simulink model "turbofan_engine_model"  (R2026b)
settings: Solver=ode45
settings Model: Creator=samjoseph  LastModifiedBy=samjoseph

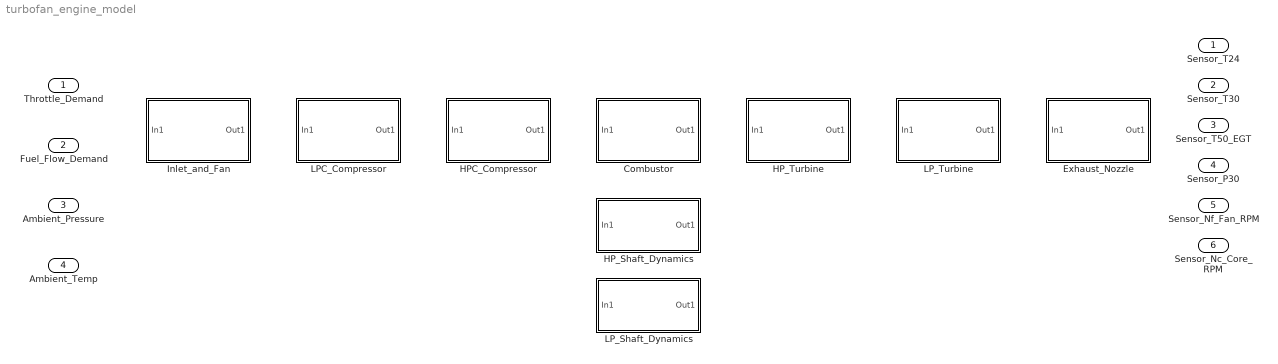
== system turbofan_engine_model ==
  Throttle_Demand : Inport
  Fuel_Flow_Demand : Inport  Port=2
  Ambient_Pressure : Inport  Port=3
  Ambient_Temp : Inport  Port=4
  Combustor : Subsystem
  Exhaust_Nozzle : Subsystem
  HPC_Compressor : Subsystem
  HP_Shaft_Dynamics : Subsystem
  HP_Turbine : Subsystem
  Inlet_and_Fan : Subsystem
  LPC_Compressor : Subsystem
  LP_Shaft_Dynamics : Subsystem
  LP_Turbine : Subsystem
  Sensor_T24 : Outport
  Sensor_T30 : Outport  Port=2
  Sensor_T50_EGT : Outport  Port=3
  Sensor_P30 : Outport  Port=4
  Sensor_Nf_Fan_RPM : Outport  Port=5
  Sensor_Nc_Core_RPM : Outport  Port=6

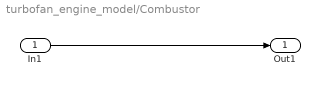
== system turbofan_engine_model/Combustor ==
  In1 : Inport
  Out1 : Outport
  wires:
  In1/1 -> Out1/1

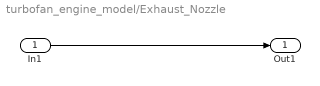
== system turbofan_engine_model/Exhaust_Nozzle ==
  In1 : Inport
  Out1 : Outport
  wires:
  In1/1 -> Out1/1

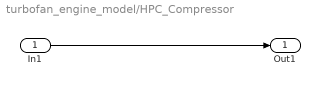
== system turbofan_engine_model/HPC_Compressor ==
  In1 : Inport
  Out1 : Outport
  wires:
  In1/1 -> Out1/1

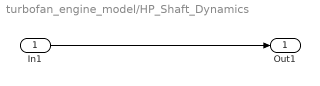
== system turbofan_engine_model/HP_Shaft_Dynamics ==
  In1 : Inport
  Out1 : Outport
  wires:
  In1/1 -> Out1/1

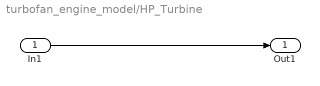
== system turbofan_engine_model/HP_Turbine ==
  In1 : Inport
  Out1 : Outport
  wires:
  In1/1 -> Out1/1

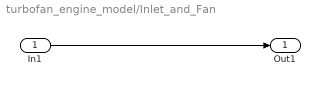
== system turbofan_engine_model/Inlet_and_Fan ==
  In1 : Inport
  Out1 : Outport
  wires:
  In1/1 -> Out1/1

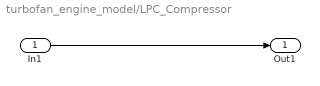
== system turbofan_engine_model/LPC_Compressor ==
  In1 : Inport
  Out1 : Outport
  wires:
  In1/1 -> Out1/1

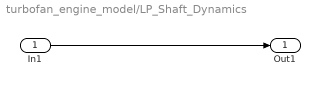
== system turbofan_engine_model/LP_Shaft_Dynamics ==
  In1 : Inport
  Out1 : Outport
  wires:
  In1/1 -> Out1/1

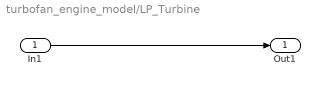
== system turbofan_engine_model/LP_Turbine ==
  In1 : Inport
  Out1 : Outport
  wires:
  In1/1 -> Out1/1
